simulink model "ESSSimulation"  (R2025a)
settings: Solver=VariableStepAuto  StartTime=0.0  StopTime=1800  RelTol=1e-3
undefined symbols (not defined in the file or in its folder): battery_builder_rtmsupport, gcbh
libraries: nesl_utility x18, P45B_98S30P_Library_lib x14, fl_lib x4, simulink x1, SignalEditorBlockLib x1
(part 1 of 8)
settings Model: Creator=saarv  LastModifiedBy=JESHNU PRANAV

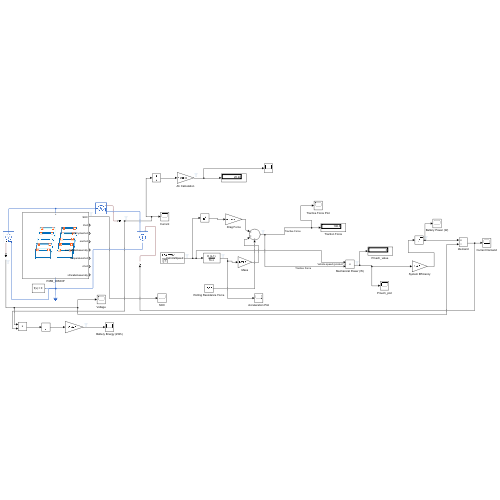
[thumbnail: Simulink's stored preview of the top-level diagram]
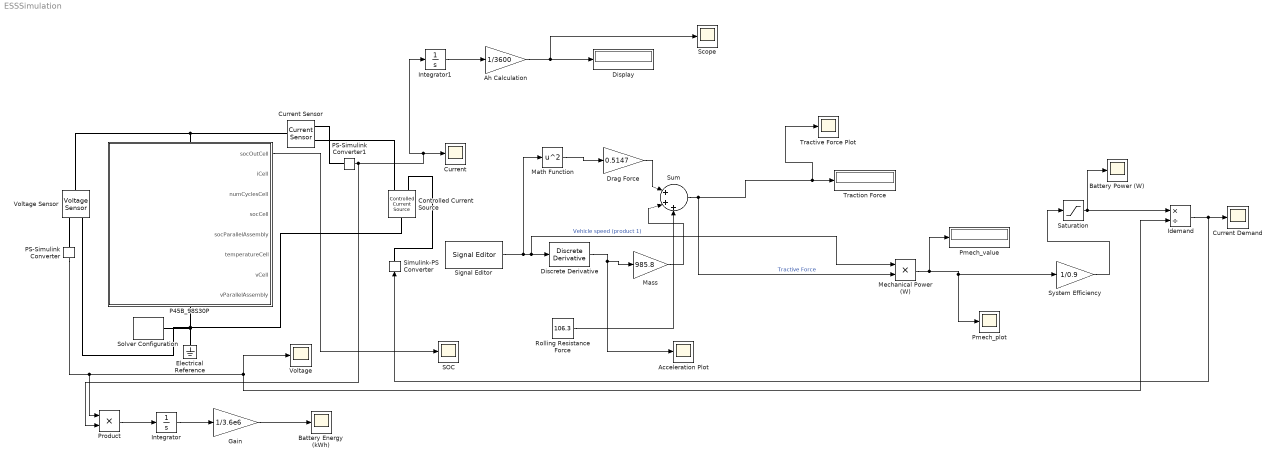
== system ESSSimulation ==
  Acceleration Plot : Scope
      settings: ActiveDisplayYMinimum=-1  ActiveDisplayYMaximum=1  DataLoggingVariableName=ScopeData3
  Ah Calculation : Gain  Gain=1/3600
  Battery Energy (kWh) : Scope
      settings: ActiveDisplayYMinimum=-0.27547832046420689  ActiveDisplayYMaximum=2.4793048841778624  DataLoggingVariableName=ScopeData8
  Battery Power (W) : Scope
      settings: ActiveDisplayYMinimum=-1660.4480803591648  ActiveDisplayYMaximum=14944.032723232487  DataLoggingVariableName=ScopeData6
  Controlled Current Source : fl_lib/Electrical/Electrical Sources/Controlled Current Source
  Current : Scope
      settings: ActiveDisplayYMinimum=-2.3494414378280619  ActiveDisplayYMaximum=21.144972940452561
  Current Demand : Scope
      settings: ActiveDisplayYMinimum=-4.1462072619256087  ActiveDisplayYMaximum=37.315865357330487  DataLoggingVariableName=ScopeData7
  Current Sensor : fl_lib/Electrical/Electrical Sensors/Current Sensor
  Discrete Derivative : simulink/Discrete/Discrete Derivative  gainval=1.0  ICPrevScaledInput=0.0  OutMin=[]  OutMax=[]  OutDataType=fixdt(1, 16)  OutScaling=2^-10  DoSatur=off
  Display : Display
  Drag Force : Gain  Gain=0.5147
  Electrical Reference : fl_lib/Electrical/Electrical Elements/Electrical Reference
  Gain : Gain  Gain=1/3.6e6
  Idemand : Product  Inputs=*/
  Integrator : Integrator
  Integrator1 : Integrator
  Mass : Gain  Gain=985.8
  Math Function : Math  Operator=square
  Mechanical Power (W) : Product
  P45B_98S30P : Subsystem  LoadFcn=battery_builder_rtmsupport('loadfcn',gcbh);
      settings: CopyFcn=battery_builder_rtmsupport('copyfcn',gcbh);  PreCopyFcn=battery_builder_rtmsupport('precopyfcn',gcbh);  PreDeleteFcn=battery_builder_rtmsupport('predeletefcn',gcbh);  PortSchema="{\"entries\":[{\"content\":{\"sides\":[{\"content\":{\"connectorIds\":[\"LConn1\"]},\"type\":\"ConnectorPlacement.EquallySpacedRectSide\",\"uuid\":\"d4e2ae1f-91bd-4f30-85c6-3b09e7a5f073\"},{\"content\":{\"connectorIds\":[\"RConn1\"],\"side\":\"RIGHT\"},\"type\":\"ConnectorPlacement.EquallySpacedRectSide\",\"uuid\":\"85839490-b33b-4096-9a8d-050120bf99f0\"},{\"content\":{\"side\":\"TOP\"},\"type\":\"ConnectorPlacement.EquallySpacedRectSide\",\"uuid\":\"ebce77ff-3da5-4228-a979-6e6121cd9cec\"},{\"content\":{\"connectorIds\":[\"Out1\",\"Out2\",\"Out3\",\"Out4\",\"Out5\",\"Out6\",\"Out7\",\"Out8\"],\"side\":\"BOTTOM\"},\"type\":\"ConnectorPlacement.EquallySpacedRectSide\",\"uuid\":\"8abbc902-ff5b-4280-b91e-4ff8c5b8e2b0\"}]},\"type\":\"ConnectorPlacement.EquallySpacedConnector\",\"uuid\":\"df0ba139-0a4a-4a35-a3e3-f1876ef380fd\"}],\"packageUris\":[\"http://schema.mathworks.com/mf0/Connector/R2020b\"],\"version\":\"1.0\"}"
      mask Display: image('$imagefile')
  PS-Simulink Converter : nesl_utility/PS-Simulink Converter  PhysicalDomain=network_engine_domain  SubClassName=ps_output  LeftPortType=input  RightPortType=output  PseudoPeriodic=off  Frequencies=[]  VectorFormat=inherit  Unit=inherit  AffineConversion=off
  PS-Simulink Converter1 : nesl_utility/PS-Simulink Converter  PhysicalDomain=network_engine_domain  SubClassName=ps_output  LeftPortType=input  RightPortType=output  PseudoPeriodic=off  Frequencies=[]  VectorFormat=inherit  Unit=inherit  AffineConversion=off
  Pmech_plot : Scope
      settings: ActiveDisplayYMinimum=-4360.824190842518  ActiveDisplayYMaximum=13768.120664078046  DataLoggingVariableName=ScopeData5
  "Pmech_value " : Display
  Product : Product
  Rolling Resistance Force : Constant  Value=106.3
  SOC : Scope
      settings: ActiveDisplayYMinimum=0.95435961378164524  ActiveDisplayYMaximum=1.0050711540242616  DataLoggingVariableName=ScopeData2
  Saturation : Saturate  UpperLimit=inf  LowerLimit=0
  Scope : Scope
      settings: ActiveDisplayYMinimum=-1  ActiveDisplayYMaximum=1  DataLoggingVariableName=ScopeData9
  Signal Editor : SignalEditorBlockLib/Signal Editor  FileName=EV_DriveProfiles.mat  ActiveScenario=SportProfile  ActiveSignal=VehicleSpeed  IsBus=off  OutputBusObjectStr=Bus: BusObject  SampleTime=10  ZeroCross=off  OutputAfterFinalValue=Setting to zero  Unit=m/s  PreserveSignalName=on  ApplySigPropsToAllScenarios=on  ApplySigPropsToAllSignals=off  SignalPropertySource=Dialog parameters
  Simulink-PS Converter : nesl_utility/Simulink-PS Converter  PhysicalDomain=network_engine_domain  SubClassName=ps_input  LeftPortType=input  RightPortType=output  PseudoPeriodic=off  Frequencies=[]  NoiseDistribution=none  NoiseParameters=[]  Unit=A  AffineConversion=off  FilteringAndDerivatives=provide  SimscapeFilterOrder=1  InputFilterTimeConstant=0.001  UdotUserProvided=0
  Solver Configuration : nesl_utility/Solver Configuration  PhysicalDomain=network_engine_domain  SubClassName=solver  LeftPortType=input  RightPortType=generic  Tones=[]  Harmonics=[]  SimulateNoise=off  Profile=off  UseLocalSampling=off  EnableSwitchedLinearOptims=on  FrequencyDomain=off  UseCCode=off  RelTol=0.001  AbsTol=0.001  MinStep=1e-09  ToWorkspace=off  RevertToSquareIcSolve=off  NumHomotopyIterations=100  PhasorMode=off  PhasorModeNumHarmonics=1  ConsistencySolver=NEWTON_XTOL_AFTER_FTOL  IndexReductionMethod=DerivativeReplacement  DoDC=off  ResidualTolerance=1e-09  ConsistencyTolSource=GLOBAL  ConsistencyAbsTol=0.001  ConsistencyRelTol=0.001  ConsistencyTolFactor=0.001  UseLocalSolver=off  LocalSolverChoice=NE_BACKWARD_EULER_ADVANCER  ResolveIndetEquations=on  FunctionEvalNumThread=1  LocalSolverSampleTime=0.001  DoFixedCost=off  MaxNonlinIter=3  MaxModeIter=2  ComputeImpulses=off  ImpulseIterations=2  LinearAlgebra=auto  LinearAlgebraNumThread=0  EquationFormulation=NE_TIME_EF  DelaysMemoryBudget=1024  AutomaticFiltering=on  FilteringTimeConstant=0.001  PartitionStorageMethod=AS_NEEDED  PartitionMemoryBudget=1024  PartitionMethod=ROBUST  MultibodyUseLocalSolver=off  MultibodyLocalSolverChoice=ODE1  MultibodyLocalSolverSampleTime=0.001
  Sum : Sum  Inputs=|+++
  System Efficiency : Gain  Gain=1/0.9
  Traction Force : Display
  Tractive Force Plot : Scope
      settings: ActiveDisplayYMinimum=-1  ActiveDisplayYMaximum=1  DataLoggingVariableName=ScopeData4
  Voltage : Scope
      settings: ActiveDisplayYMinimum=398.6789246794516  ActiveDisplayYMaximum=409.58498614672749
  Voltage Sensor : fl_lib/Electrical/Electrical Sensors/Voltage Sensor
  wires:
  PS-Simulink Converter/1 -> Product/1, Idemand/2, Voltage/1
  PS-Simulink Converter1/1 -> Product/2, Integrator1/1, Current/1
  P45B_98S30P/1(socOutCell) -> SOC/1
  Signal Editor/1 -> Math Function/1, Discrete Derivative/1, Mechanical Power (W)/1  "Vehicle speed (product 1)"
  Math Function/1 -> Drag Force/1
  Discrete Derivative/1 -> Acceleration Plot/1, Mass/1
  Drag Force/1 -> Sum/1
  Mass/1 -> Sum/2
  Rolling Resistance Force/1 -> Sum/3
  Sum/1 -> Mechanical Power (W)/2, Tractive Force Plot/1, Traction Force/1  "Tractive Force"
  Mechanical Power (W)/1 -> System Efficiency/1, Pmech_plot/1, "Pmech_value "/1
  System Efficiency/1 -> Saturation/1
  Saturation/1 -> Idemand/1, Battery Power (W)/1
  Idemand/1 -> Simulink-PS Converter/1, Current Demand/1
  Product/1 -> Integrator/1
  Integrator/1 -> Gain/1
  Gain/1 -> Battery Energy (kWh)/1
  Integrator1/1 -> Ah Calculation/1
  Ah Calculation/1 -> Scope/1, Display/1
  connections:
  Voltage Sensor/LConn1 -- Current Sensor/LConn1 -- P45B_98S30P/LConn1
  Electrical Reference/LConn1 -- P45B_98S30P/RConn1 -- Controlled Current Source/LConn1 -- Voltage Sensor/RConn2 -- Solver Configuration/RConn1
  Simulink-PS Converter/RConn1 -- Controlled Current Source/RConn1
  Voltage Sensor/RConn1 -- PS-Simulink Converter/LConn1
  Current Sensor/RConn1 -- PS-Simulink Converter1/LConn1
  Controlled Current Source/RConn2 -- Current Sensor/RConn2

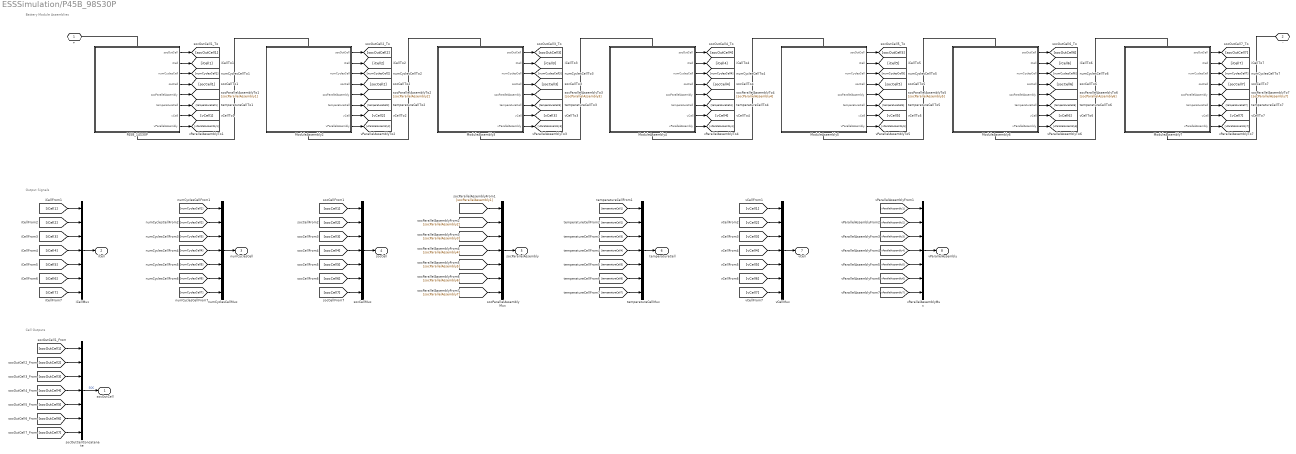
== system ESSSimulation/P45B_98S30P ==
  note: Cell Outputs
  note: Output Signals
  note: Battery Module Assemblies
  ModuleAssembly2 : Subsystem  LoadFcn=battery_builder_rtmsupport('loadfcn',gcbh);
      settings: CopyFcn=battery_builder_rtmsupport('copyfcn',gcbh);  PreCopyFcn=battery_builder_rtmsupport('precopyfcn',gcbh);  PreDeleteFcn=battery_builder_rtmsupport('predeletefcn',gcbh);  PortSchema="{\"entries\":[{\"content\":{\"sides\":[{\"content\":{\"connectorIds\":[\"LConn1\"]},\"type\":\"ConnectorPlacement.EquallySpacedRectSide\",\"uuid\":\"d4e2ae1f-91bd-4f30-85c6-3b09e7a5f073\"},{\"content\":{\"connectorIds\":[\"RConn1\"],\"side\":\"RIGHT\"},\"type\":\"ConnectorPlacement.EquallySpacedRectSide\",\"uuid\":\"85839490-b33b-4096-9a8d-050120bf99f0\"},{\"content\":{\"side\":\"TOP\"},\"type\":\"ConnectorPlacement.EquallySpacedRectSide\",\"uuid\":\"ebce77ff-3da5-4228-a979-6e6121cd9cec\"},{\"content\":{\"connectorIds\":[\"Out1\",\"Out2\",\"Out3\",\"Out4\",\"Out5\",\"Out6\",\"Out7\",\"Out8\"],\"side\":\"BOTTOM\"},\"type\":\"ConnectorPlacement.EquallySpacedRectSide\",\"uuid\":\"bb73c3c7-4a19-4c53-8f91-0cca065a4ce2\"}]},\"type\":\"ConnectorPlacement.EquallySpacedConnector\",\"uuid\":\"df0ba139-0a4a-4a35-a3e3-f1876ef380fd\"}],\"packageUris\":[\"http://schema.mathworks.com/mf0/Connector/R2020b\"],\"version\":\"1.0\"}"
      mask Display: image('$imagefile')
  ModuleAssembly3 : Subsystem  LoadFcn=battery_builder_rtmsupport('loadfcn',gcbh);
      settings: CopyFcn=battery_builder_rtmsupport('copyfcn',gcbh);  PreCopyFcn=battery_builder_rtmsupport('precopyfcn',gcbh);  PreDeleteFcn=battery_builder_rtmsupport('predeletefcn',gcbh);  PortSchema="{\"entries\":[{\"content\":{\"sides\":[{\"content\":{\"connectorIds\":[\"LConn1\"]},\"type\":\"ConnectorPlacement.EquallySpacedRectSide\",\"uuid\":\"d4e2ae1f-91bd-4f30-85c6-3b09e7a5f073\"},{\"content\":{\"connectorIds\":[\"RConn1\"],\"side\":\"RIGHT\"},\"type\":\"ConnectorPlacement.EquallySpacedRectSide\",\"uuid\":\"85839490-b33b-4096-9a8d-050120bf99f0\"},{\"content\":{\"side\":\"TOP\"},\"type\":\"ConnectorPlacement.EquallySpacedRectSide\",\"uuid\":\"ebce77ff-3da5-4228-a979-6e6121cd9cec\"},{\"content\":{\"connectorIds\":[\"Out1\",\"Out2\",\"Out3\",\"Out4\",\"Out5\",\"Out6\",\"Out7\",\"Out8\"],\"side\":\"BOTTOM\"},\"type\":\"ConnectorPlacement.EquallySpacedRectSide\",\"uuid\":\"bb73c3c7-4a19-4c53-8f91-0cca065a4ce2\"}]},\"type\":\"ConnectorPlacement.EquallySpacedConnector\",\"uuid\":\"df0ba139-0a4a-4a35-a3e3-f1876ef380fd\"}],\"packageUris\":[\"http://schema.mathworks.com/mf0/Connector/R2020b\"],\"version\":\"1.0\"}"
      mask Display: image('moduleAssembly_1.JPG');
  ModuleAssembly4 : Subsystem  LoadFcn=battery_builder_rtmsupport('loadfcn',gcbh);
      settings: CopyFcn=battery_builder_rtmsupport('copyfcn',gcbh);  PreCopyFcn=battery_builder_rtmsupport('precopyfcn',gcbh);  PreDeleteFcn=battery_builder_rtmsupport('predeletefcn',gcbh);  PortSchema="{\"entries\":[{\"content\":{\"sides\":[{\"content\":{\"connectorIds\":[\"LConn1\"]},\"type\":\"ConnectorPlacement.EquallySpacedRectSide\",\"uuid\":\"d4e2ae1f-91bd-4f30-85c6-3b09e7a5f073\"},{\"content\":{\"connectorIds\":[\"RConn1\"],\"side\":\"RIGHT\"},\"type\":\"ConnectorPlacement.EquallySpacedRectSide\",\"uuid\":\"85839490-b33b-4096-9a8d-050120bf99f0\"},{\"content\":{\"side\":\"TOP\"},\"type\":\"ConnectorPlacement.EquallySpacedRectSide\",\"uuid\":\"ebce77ff-3da5-4228-a979-6e6121cd9cec\"},{\"content\":{\"connectorIds\":[\"Out1\",\"Out2\",\"Out3\",\"Out4\",\"Out5\",\"Out6\",\"Out7\",\"Out8\"],\"side\":\"BOTTOM\"},\"type\":\"ConnectorPlacement.EquallySpacedRectSide\",\"uuid\":\"bb73c3c7-4a19-4c53-8f91-0cca065a4ce2\"}]},\"type\":\"ConnectorPlacement.EquallySpacedConnector\",\"uuid\":\"df0ba139-0a4a-4a35-a3e3-f1876ef380fd\"}],\"packageUris\":[\"http://schema.mathworks.com/mf0/Connector/R2020b\"],\"version\":\"1.0\"}"
      mask Display: image('moduleAssembly_2.JPG');
  ModuleAssembly5 : Subsystem  LoadFcn=battery_builder_rtmsupport('loadfcn',gcbh);
      settings: CopyFcn=battery_builder_rtmsupport('copyfcn',gcbh);  PreCopyFcn=battery_builder_rtmsupport('precopyfcn',gcbh);  PreDeleteFcn=battery_builder_rtmsupport('predeletefcn',gcbh);  PortSchema="{\"entries\":[{\"content\":{\"sides\":[{\"content\":{\"connectorIds\":[\"LConn1\"]},\"type\":\"ConnectorPlacement.EquallySpacedRectSide\",\"uuid\":\"d4e2ae1f-91bd-4f30-85c6-3b09e7a5f073\"},{\"content\":{\"connectorIds\":[\"RConn1\"],\"side\":\"RIGHT\"},\"type\":\"ConnectorPlacement.EquallySpacedRectSide\",\"uuid\":\"85839490-b33b-4096-9a8d-050120bf99f0\"},{\"content\":{\"side\":\"TOP\"},\"type\":\"ConnectorPlacement.EquallySpacedRectSide\",\"uuid\":\"ebce77ff-3da5-4228-a979-6e6121cd9cec\"},{\"content\":{\"connectorIds\":[\"Out1\",\"Out2\",\"Out3\",\"Out4\",\"Out5\",\"Out6\",\"Out7\",\"Out8\"],\"side\":\"BOTTOM\"},\"type\":\"ConnectorPlacement.EquallySpacedRectSide\",\"uuid\":\"bb73c3c7-4a19-4c53-8f91-0cca065a4ce2\"}]},\"type\":\"ConnectorPlacement.EquallySpacedConnector\",\"uuid\":\"df0ba139-0a4a-4a35-a3e3-f1876ef380fd\"}],\"packageUris\":[\"http://schema.mathworks.com/mf0/Connector/R2020b\"],\"version\":\"1.0\"}"
      mask Display: image('moduleAssembly_3.JPG');
  ModuleAssembly6 : Subsystem  LoadFcn=battery_builder_rtmsupport('loadfcn',gcbh);
      settings: CopyFcn=battery_builder_rtmsupport('copyfcn',gcbh);  PreCopyFcn=battery_builder_rtmsupport('precopyfcn',gcbh);  PreDeleteFcn=battery_builder_rtmsupport('predeletefcn',gcbh);  PortSchema="{\"entries\":[{\"content\":{\"sides\":[{\"content\":{\"connectorIds\":[\"LConn1\"]},\"type\":\"ConnectorPlacement.EquallySpacedRectSide\",\"uuid\":\"d4e2ae1f-91bd-4f30-85c6-3b09e7a5f073\"},{\"content\":{\"connectorIds\":[\"RConn1\"],\"side\":\"RIGHT\"},\"type\":\"ConnectorPlacement.EquallySpacedRectSide\",\"uuid\":\"85839490-b33b-4096-9a8d-050120bf99f0\"},{\"content\":{\"side\":\"TOP\"},\"type\":\"ConnectorPlacement.EquallySpacedRectSide\",\"uuid\":\"ebce77ff-3da5-4228-a979-6e6121cd9cec\"},{\"content\":{\"connectorIds\":[\"Out1\",\"Out2\",\"Out3\",\"Out4\",\"Out5\",\"Out6\",\"Out7\",\"Out8\"],\"side\":\"BOTTOM\"},\"type\":\"ConnectorPlacement.EquallySpacedRectSide\",\"uuid\":\"bb73c3c7-4a19-4c53-8f91-0cca065a4ce2\"}]},\"type\":\"ConnectorPlacement.EquallySpacedConnector\",\"uuid\":\"df0ba139-0a4a-4a35-a3e3-f1876ef380fd\"}],\"packageUris\":[\"http://schema.mathworks.com/mf0/Connector/R2020b\"],\"version\":\"1.0\"}"
      mask Display: image('moduleAssembly_4.JPG');
  ModuleAssembly7 : Subsystem  LoadFcn=battery_builder_rtmsupport('loadfcn',gcbh);
      settings: CopyFcn=battery_builder_rtmsupport('copyfcn',gcbh);  PreCopyFcn=battery_builder_rtmsupport('precopyfcn',gcbh);  PreDeleteFcn=battery_builder_rtmsupport('predeletefcn',gcbh);  PortSchema="{\"entries\":[{\"content\":{\"sides\":[{\"content\":{\"connectorIds\":[\"LConn1\"]},\"type\":\"ConnectorPlacement.EquallySpacedRectSide\",\"uuid\":\"d4e2ae1f-91bd-4f30-85c6-3b09e7a5f073\"},{\"content\":{\"connectorIds\":[\"RConn1\"],\"side\":\"RIGHT\"},\"type\":\"ConnectorPlacement.EquallySpacedRectSide\",\"uuid\":\"85839490-b33b-4096-9a8d-050120bf99f0\"},{\"content\":{\"side\":\"TOP\"},\"type\":\"ConnectorPlacement.EquallySpacedRectSide\",\"uuid\":\"ebce77ff-3da5-4228-a979-6e6121cd9cec\"},{\"content\":{\"connectorIds\":[\"Out1\",\"Out2\",\"Out3\",\"Out4\",\"Out5\",\"Out6\",\"Out7\",\"Out8\"],\"side\":\"BOTTOM\"},\"type\":\"ConnectorPlacement.EquallySpacedRectSide\",\"uuid\":\"bb73c3c7-4a19-4c53-8f91-0cca065a4ce2\"}]},\"type\":\"ConnectorPlacement.EquallySpacedConnector\",\"uuid\":\"df0ba139-0a4a-4a35-a3e3-f1876ef380fd\"}],\"packageUris\":[\"http://schema.mathworks.com/mf0/Connector/R2020b\"],\"version\":\"1.0\"}"
      mask Display: image('moduleAssembly_5.JPG');
  P45B_14S30P : Subsystem  LoadFcn=battery_builder_rtmsupport('loadfcn',gcbh);
      settings: CopyFcn=battery_builder_rtmsupport('copyfcn',gcbh);  PreCopyFcn=battery_builder_rtmsupport('precopyfcn',gcbh);  PreDeleteFcn=battery_builder_rtmsupport('predeletefcn',gcbh);  PortSchema="{\"entries\":[{\"content\":{\"sides\":[{\"content\":{\"connectorIds\":[\"LConn1\"]},\"type\":\"ConnectorPlacement.EquallySpacedRectSide\",\"uuid\":\"d4e2ae1f-91bd-4f30-85c6-3b09e7a5f073\"},{\"content\":{\"connectorIds\":[\"RConn1\"],\"side\":\"RIGHT\"},\"type\":\"ConnectorPlacement.EquallySpacedRectSide\",\"uuid\":\"85839490-b33b-4096-9a8d-050120bf99f0\"},{\"content\":{\"side\":\"TOP\"},\"type\":\"ConnectorPlacement.EquallySpacedRectSide\",\"uuid\":\"ebce77ff-3da5-4228-a979-6e6121cd9cec\"},{\"content\":{\"connectorIds\":[\"Out1\",\"Out2\",\"Out3\",\"Out4\",\"Out5\",\"Out6\",\"Out7\",\"Out8\"],\"side\":\"BOTTOM\"},\"type\":\"ConnectorPlacement.EquallySpacedRectSide\",\"uuid\":\"bb73c3c7-4a19-4c53-8f91-0cca065a4ce2\"}]},\"type\":\"ConnectorPlacement.EquallySpacedConnector\",\"uuid\":\"df0ba139-0a4a-4a35-a3e3-f1876ef380fd\"}],\"packageUris\":[\"http://schema.mathworks.com/mf0/Connector/R2020b\"],\"version\":\"1.0\"}"
      mask Display: image('moduleAssembly_6.JPG');
  iCellMux : Mux  Inputs=7
  numCyclesCellMux : Mux  Inputs=7
  socCellMux : Mux  Inputs=7
  socOutCellConcatenate : Concatenate  NumInputs=7  Mode=Multidimensional array  ConcatenateDimension=2
  socParallelAssemblyMux : Mux  Inputs=7
  temperatureCellMux : Mux  Inputs=7
  vCellMux : Mux  Inputs=7
  vParallelAssemblyMux : Mux  Inputs=7
  + : PMIOPort  Side=Left
  - : PMIOPort  Port=2  Side=Right
  socOutCell : Outport
  iCell : Outport  Port=2
  numCyclesCell : Outport  Port=3
  socCell : Outport  Port=4
  socParallelAssembly : Outport  Port=5
  temperatureCell : Outport  Port=6
  vCell : Outport  Port=7
  vParallelAssembly : Outport  Port=8
  wires:
  ModuleAssembly7/1(socOutCell) -> [socOutCell7]
  ModuleAssembly6/1(socOutCell) -> [socOutCell6]
  ModuleAssembly5/1(socOutCell) -> [socOutCell5]
  ModuleAssembly4/1(socOutCell) -> [socOutCell4]
  ModuleAssembly3/1(socOutCell) -> [socOutCell3]
  ModuleAssembly2/1(socOutCell) -> [socOutCell2]
  P45B_14S30P/1(socOutCell) -> [socOutCell1]
  [vParallelAssembly7] -> vParallelAssemblyMux/7
  ModuleAssembly7/8(vParallelAssembly) -> [vParallelAssembly7]
  [vCell7] -> vCellMux/7
  ModuleAssembly7/7(vCell) -> [vCell7]
  [temperatureCell7] -> temperatureCellMux/7
  ModuleAssembly7/6(temperatureCell) -> [temperatureCell7]
  [socParallelAssembly7] -> socParallelAssemblyMux/7
  ModuleAssembly7/5(socParallelAssembly) -> [socParallelAssembly7]
  [socCell7] -> socCellMux/7
  ModuleAssembly7/4(socCell) -> [socCell7]
  [numCyclesCell7] -> numCyclesCellMux/7
  ModuleAssembly7/3(numCyclesCell) -> [numCyclesCell7]
  [iCell7] -> iCellMux/7
  ModuleAssembly7/2(iCell) -> [iCell7]
  [vParallelAssembly6] -> vParallelAssemblyMux/6
  ModuleAssembly6/8(vParallelAssembly) -> [vParallelAssembly6]
  [vCell6] -> vCellMux/6
  ModuleAssembly6/7(vCell) -> [vCell6]
  [temperatureCell6] -> temperatureCellMux/6
  ModuleAssembly6/6(temperatureCell) -> [temperatureCell6]
  [socParallelAssembly6] -> socParallelAssemblyMux/6
  ModuleAssembly6/5(socParallelAssembly) -> [socParallelAssembly6]
  [socCell6] -> socCellMux/6
  ModuleAssembly6/4(socCell) -> [socCell6]
  [numCyclesCell6] -> numCyclesCellMux/6
  ModuleAssembly6/3(numCyclesCell) -> [numCyclesCell6]
  [iCell6] -> iCellMux/6
  ModuleAssembly6/2(iCell) -> [iCell6]
  [vParallelAssembly5] -> vParallelAssemblyMux/5
  ModuleAssembly5/8(vParallelAssembly) -> [vParallelAssembly5]
  [vCell5] -> vCellMux/5
  ModuleAssembly5/7(vCell) -> [vCell5]
  [temperatureCell5] -> temperatureCellMux/5
  ModuleAssembly5/6(temperatureCell) -> [temperatureCell5]
  [socParallelAssembly5] -> socParallelAssemblyMux/5
  ModuleAssembly5/5(socParallelAssembly) -> [socParallelAssembly5]
  [socCell5] -> socCellMux/5
  ModuleAssembly5/4(socCell) -> [socCell5]
  [numCyclesCell5] -> numCyclesCellMux/5
  ModuleAssembly5/3(numCyclesCell) -> [numCyclesCell5]
  [iCell5] -> iCellMux/5
  ModuleAssembly5/2(iCell) -> [iCell5]
  [vParallelAssembly4] -> vParallelAssemblyMux/4
  ModuleAssembly4/8(vParallelAssembly) -> [vParallelAssembly4]
  [vCell4] -> vCellMux/4
  ModuleAssembly4/7(vCell) -> [vCell4]
  [temperatureCell4] -> temperatureCellMux/4
  ModuleAssembly4/6(temperatureCell) -> [temperatureCell4]
  [socParallelAssembly4] -> socParallelAssemblyMux/4
  ModuleAssembly4/5(socParallelAssembly) -> [socParallelAssembly4]
  [socCell4] -> socCellMux/4
  ModuleAssembly4/4(socCell) -> [socCell4]
  [numCyclesCell4] -> numCyclesCellMux/4
  ModuleAssembly4/3(numCyclesCell) -> [numCyclesCell4]
  [iCell4] -> iCellMux/4
  ModuleAssembly4/2(iCell) -> [iCell4]
  [vParallelAssembly3] -> vParallelAssemblyMux/3
  ModuleAssembly3/8(vParallelAssembly) -> [vParallelAssembly3]
  [vCell3] -> vCellMux/3
  ModuleAssembly3/7(vCell) -> [vCell3]
  [temperatureCell3] -> temperatureCellMux/3
  ModuleAssembly3/6(temperatureCell) -> [temperatureCell3]
  [socParallelAssembly3] -> socParallelAssemblyMux/3
  ModuleAssembly3/5(socParallelAssembly) -> [socParallelAssembly3]
  [socCell3] -> socCellMux/3
  ModuleAssembly3/4(socCell) -> [socCell3]
  [numCyclesCell3] -> numCyclesCellMux/3
  ModuleAssembly3/3(numCyclesCell) -> [numCyclesCell3]
  [iCell3] -> iCellMux/3
  ModuleAssembly3/2(iCell) -> [iCell3]
  [vParallelAssembly2] -> vParallelAssemblyMux/2
  ModuleAssembly2/8(vParallelAssembly) -> [vParallelAssembly2]
  [vCell2] -> vCellMux/2
  ModuleAssembly2/7(vCell) -> [vCell2]
  [temperatureCell2] -> temperatureCellMux/2
  ModuleAssembly2/6(temperatureCell) -> [temperatureCell2]
  [socParallelAssembly2] -> socParallelAssemblyMux/2
  ModuleAssembly2/5(socParallelAssembly) -> [socParallelAssembly2]
  [socCell2] -> socCellMux/2
  ModuleAssembly2/4(socCell) -> [socCell2]
  [numCyclesCell2] -> numCyclesCellMux/2
  ModuleAssembly2/3(numCyclesCell) -> [numCyclesCell2]
  [iCell2] -> iCellMux/2
  ModuleAssembly2/2(iCell) -> [iCell2]
  [vParallelAssembly1] -> vParallelAssemblyMux/1
  vParallelAssemblyMux/1 -> vParallelAssembly/1
  P45B_14S30P/8(vParallelAssembly) -> [vParallelAssembly1]
  [vCell1] -> vCellMux/1
  vCellMux/1 -> vCell/1
  P45B_14S30P/7(vCell) -> [vCell1]
  [temperatureCell1] -> temperatureCellMux/1
  temperatureCellMux/1 -> temperatureCell/1
  P45B_14S30P/6(temperatureCell) -> [temperatureCell1]
  [socParallelAssembly1] -> socParallelAssemblyMux/1
  socParallelAssemblyMux/1 -> socParallelAssembly/1
  P45B_14S30P/5(socParallelAssembly) -> [socParallelAssembly1]
  [socCell1] -> socCellMux/1
  socCellMux/1 -> socCell/1
  P45B_14S30P/4(socCell) -> [socCell1]
  [numCyclesCell1] -> numCyclesCellMux/1
  numCyclesCellMux/1 -> numCyclesCell/1
  P45B_14S30P/3(numCyclesCell) -> [numCyclesCell1]
  [iCell1] -> iCellMux/1
  iCellMux/1 -> iCell/1
  P45B_14S30P/2(iCell) -> [iCell1]
  [socOutCell7] -> socOutCellConcatenate/7
  [socOutCell6] -> socOutCellConcatenate/6
  [socOutCell5] -> socOutCellConcatenate/5
  [socOutCell4] -> socOutCellConcatenate/4
  [socOutCell3] -> socOutCellConcatenate/3
  [socOutCell2] -> socOutCellConcatenate/2
  [socOutCell1] -> socOutCellConcatenate/1
  socOutCellConcatenate/1 -> socOutCell/1  "SOC"
  connections:
  ModuleAssembly7/RConn1 -- -/RConn1
  P45B_14S30P/LConn1 -- +/RConn1
  ModuleAssembly7/LConn1 -- ModuleAssembly6/RConn1
  ModuleAssembly6/LConn1 -- ModuleAssembly5/RConn1
  ModuleAssembly5/LConn1 -- ModuleAssembly4/RConn1
  ModuleAssembly4/LConn1 -- ModuleAssembly3/RConn1
  ModuleAssembly3/LConn1 -- ModuleAssembly2/RConn1
  ModuleAssembly2/LConn1 -- P45B_14S30P/RConn1
